simulink model "gfm_battery_sil"  (R2018b)
settings: Solver=ode45  StartTime=0.0  StopTime=100  RelTol=1e-3
PreLoadFcn:
  | load_system('../simulink_reference_models/test_sequence_lib');
  | load_system('../simulink_reference_models/controls_element_lib');
InitFcn:
  | close all;
  | clear all;
  | clc;
  | 
  | % frequency nominals
  | F_NOM = 60;
  | W_NOM = 2 * pi * F_NOM;
  | 
  | % base values relative to inverter
  | % --------------------------------
  | VLL_INV_NOM = 480;
  | P_INV_NOM = 1e6;
  | Q_INV_NOM = 0.5e6;
  | S_INV_NOM = sqrt(P_INV_NOM^2 + Q_INV_NOM^2);
  | 
  | I_INV_BASE = S_INV_NOM/(sqrt(3)*VLL_INV_NOM);
  | Z_INV_BASE = VLL_INV_NOM^2/S_INV_NOM;
  | L_INV_BASE = Z_INV_BASE / W_NOM;
  | C_INV_BASE = 1 / (Z_INV_BASE * W_NOM);
  | 
  | % nominal ratings for power system model
  | % --------------------------------------
  | INVERTER_COUNT = 100;
  | 
  | VLV_NOM = VLL_INV_NOM;
  | VMV_NOM = 35e3;
  | VHV_NOM = 230e3;
  | S_PLANT = INVERTER_COUNT * S_INV_NOM;
  | 
  | N_GSU = VHV_NOM/VMV_NOM;
  | N_MVT = VMV_NOM/VLV_NOM;
  | 
  | I_LV_BASE = S_PLANT/(sqrt(3)*VLV_NOM);
  | I_MV_BASE = S_PLANT/(sqrt(3)*VMV_NOM);
  | I_HV_BASE = S_PLANT/(sqrt(3)*VHV_NOM);
  | 
  | Z_LV_BASE = VLV_NOM^2/S_PLANT;
  | Z_MV_BASE = VMV_NOM^2/S_PLANT;
  | Z_HV_BASE = VHV_NOM^2/S_PLANT;
  | 
  | L_LV_BASE = Z_LV_BASE / W_NOM;
  | L_MV_BASE = Z_MV_BASE / W_NOM;
  | L_HV_BASE = Z_HV_BASE / W_NOM;
  | C_LV_BASE = 1 / (Z_LV_BASE * W_NOM);
  | C_MV_BASE = 1 / (Z_MV_BASE * W_NOM);
  | C_HV_BASE = 1 / (Z_HV_BASE * W_NOM);
libraries: test_sequence_lib x11, controls_element_lib x2
settings Model: SimulationMode=accelerator  Creator=HussamAlatrash  LastModifiedBy=ahhei
settings DataIOCC: ReturnWorkspaceOutputs=on
settings DebuggingCC: UnconnectedInputMsg=none  UnconnectedOutputMsg=none  UnconnectedLineMsg=none
settings ModelReferenceCC: EnableRefExpFcnMdlSchedulingChecks=off
settings RTWCC: Description=Generic Real-Time Target
settings ConfigComp: CovBoundaryAbsTol=1.0e-5

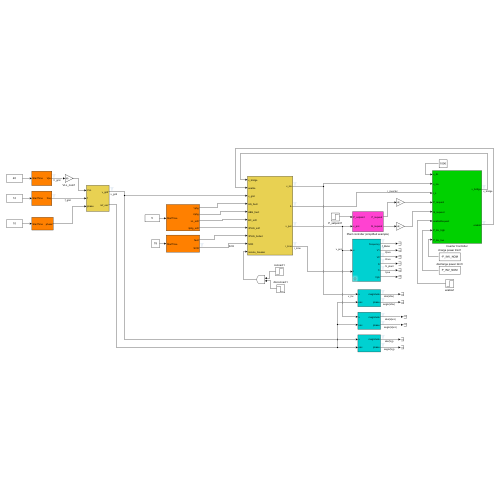
[thumbnail: Simulink's stored preview of the top-level diagram]
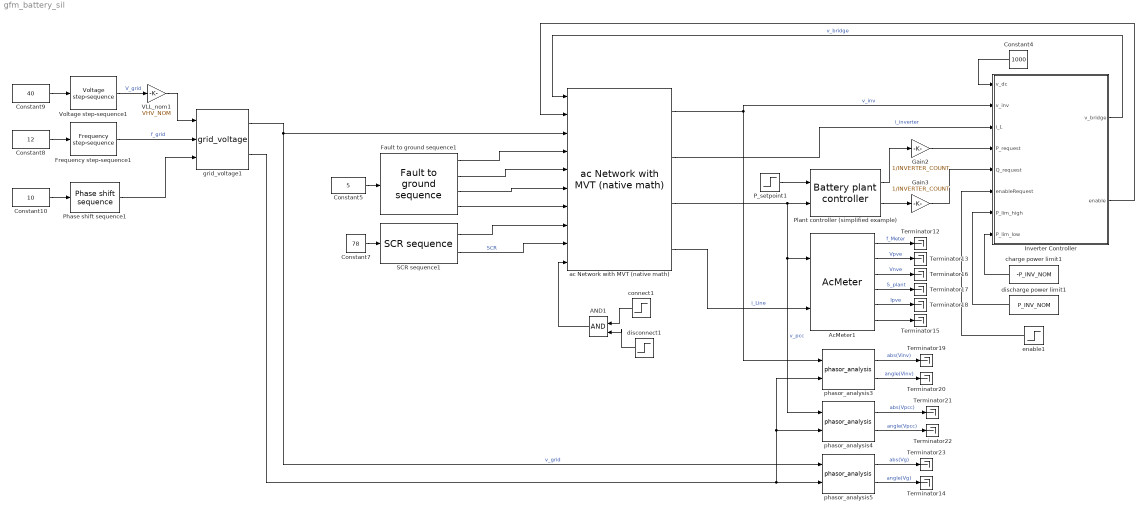
== system gfm_battery_sil ==
  AND1 : Logic  IconShape=distinctive  AllPortsSameDT=off  OutDataTypeStr=boolean
  AcMeter1 : test_sequence_lib/AcMeter  VllRated=VHV_NOM
  Constant10 : Constant  Value=10
  Constant4 : Constant  Value=1000
  Constant5 : Constant  Value=5
  Constant7 : Constant  Value=78
  Constant8 : Constant  Value=12
  Constant9 : Constant  Value=40
  Fault to ground sequence1 : test_sequence_lib/Fault to ground sequence  SystemSampleTime=-1  EmptyChoice=off  PassThrough=off  PassThroughVariantControl=(default)  EmptyChoiceVariantControl=(default)  Latency=0  AutoFrameSizeCalculation=off
  Frequency step-sequence1 : test_sequence_lib/Frequency step-sequence  SystemSampleTime=-1  EmptyChoice=off  PassThrough=off  PassThroughVariantControl=(default)  EmptyChoiceVariantControl=(default)  Latency=0  AutoFrameSizeCalculation=off
  Gain2 : Gain  Gain=1/INVERTER_COUNT
  Gain3 : Gain  Gain=1/INVERTER_COUNT
  Inverter Controller : Subsystem
  P_setpoint1 : Step  Time=4  After=S_PLANT*0.5  SampleTime=0
  Phase shift sequence1 : test_sequence_lib/Phase shift sequence  SystemSampleTime=-1  EmptyChoice=off  PassThrough=off  PassThroughVariantControl=(default)  EmptyChoiceVariantControl=(default)  Latency=0  AutoFrameSizeCalculation=off
  Plant controller (simplified example) : controls_element_lib/Battery plant controller  SystemSampleTime=-1  EmptyChoice=off  PassThrough=off  PassThroughVariantControl=(default)  EmptyChoiceVariantControl=(default)  Latency=0  AutoFrameSizeCalculation=off
  SCR sequence1 : test_sequence_lib/SCR sequence  SystemSampleTime=-1  EmptyChoice=off  PassThrough=off  PassThroughVariantControl=(default)  EmptyChoiceVariantControl=(default)  Latency=0  AutoFrameSizeCalculation=off
  Terminator{12..23} (12 alike) : Terminator
  VLL_nom1 : Gain  Gain=VHV_NOM
  Voltage step-sequence1 : test_sequence_lib/Voltage step-sequence  SystemSampleTime=-1  EmptyChoice=off  PassThrough=off  PassThroughVariantControl=(default)  EmptyChoiceVariantControl=(default)  Latency=0  AutoFrameSizeCalculation=off
  ac Network with MVT (native math) : test_sequence_lib/ac Network with MVT (native math)  SystemSampleTime=-1  EmptyChoice=off  PassThrough=off  PassThroughVariantControl=(default)  EmptyChoiceVariantControl=(default)  Latency=0  AutoFrameSizeCalculation=off
  charge power limit1 : Constant  Value=-P_INV_NOM
  connect1 : Step  Time=0  SampleTime=0
  discharge power limit1 : Constant  Value=P_INV_NOM
  disconnect1 : Step  Time=97  Before=1  After=0  SampleTime=0
  enable1 : Step  Time=0.5  SampleTime=0
  grid_voltage1 : test_sequence_lib/grid_voltage  SystemSampleTime=-1  EmptyChoice=off  PassThrough=off  PassThroughVariantControl=(default)  EmptyChoiceVariantControl=(default)  Latency=0  AutoFrameSizeCalculation=off
  phasor_analysis3 : test_sequence_lib/phasor_analysis  SystemSampleTime=-1  EmptyChoice=off  PassThrough=off  PassThroughVariantControl=(default)  EmptyChoiceVariantControl=(default)  Latency=0  AutoFrameSizeCalculation=off
  phasor_analysis4 : test_sequence_lib/phasor_analysis  SystemSampleTime=-1  EmptyChoice=off  PassThrough=off  PassThroughVariantControl=(default)  EmptyChoiceVariantControl=(default)  Latency=0  AutoFrameSizeCalculation=off
  phasor_analysis5 : test_sequence_lib/phasor_analysis  SystemSampleTime=-1  EmptyChoice=off  PassThrough=off  PassThroughVariantControl=(default)  EmptyChoiceVariantControl=(default)  Latency=0  AutoFrameSizeCalculation=off
  wires:
  Voltage step-sequence1/1 -> VLL_nom1/1  "V_grid"
  Constant9/1 -> Voltage step-sequence1/1
  Fault to ground sequence1/2 -> ac Network with MVT (native math)/5
  AND1/1 -> ac Network with MVT (native math)/10
  Constant4/1 -> Inverter Controller/1(v_dc)
  Constant10/1 -> Phase shift sequence1/1
  AcMeter1/3 -> Terminator16/1  "Vnve"
  discharge power limit1/1 -> Inverter Controller/7(P_lim_high)
  Fault to ground sequence1/3 -> ac Network with MVT (native math)/6
  AcMeter1/6 -> Terminator15/1
  Inverter Controller/1(v_bridge) -> ac Network with MVT (native math)/1  "v_bridge"
  Constant7/1 -> SCR sequence1/1
  AcMeter1/2 -> Terminator13/1  "Vpve"
  Plant controller (simplified example)/1 -> Gain2/1
  ac Network with MVT (native math)/1 -> Inverter Controller/2(v_inv), phasor_analysis3/1  "v_inv"
  Constant5/1 -> Fault to ground sequence1/1
  P_setpoint1/1 -> Plant controller (simplified example)/1
  phasor_analysis5/1 -> Terminator23/1  "abs(Vg)"
  AcMeter1/5 -> Terminator18/1  "Ipve"
  Gain3/1 -> Inverter Controller/5(Q_request)
  Plant controller (simplified example)/2 -> Gain3/1
  grid_voltage1/1 -> ac Network with MVT (native math)/3, phasor_analysis5/1  "v_grid"
  phasor_analysis4/2 -> Terminator22/1  "angle(Vpcc)"
  SCR sequence1/1 -> ac Network with MVT (native math)/8
  phasor_analysis3/1 -> Terminator19/1  "abs(Vinv)"
  Phase shift sequence1/1 -> grid_voltage1/3
  AcMeter1/4 -> Terminator17/1  "S_plant"
  ac Network with MVT (native math)/4 -> AcMeter1/2  "i_Line"
  AcMeter1/1 -> Terminator12/1  "f_Meter"
  VLL_nom1/1 -> grid_voltage1/1
  phasor_analysis3/2 -> Terminator20/1  "angle(Vinv)"
  SCR sequence1/2 -> ac Network with MVT (native math)/9  "SCR"
  ac Network with MVT (native math)/2 -> Inverter Controller/3(i_L)  "i_inverter"
  disconnect1/1 -> AND1/2
  Fault to ground sequence1/4 -> ac Network with MVT (native math)/7
  Gain2/1 -> Inverter Controller/4(P_request)
  ac Network with MVT (native math)/3 -> Plant controller (simplified example)/2, phasor_analysis4/1, AcMeter1/1  "v_pcc"
  charge power limit1/1 -> Inverter Controller/8(P_lim_low)
  Inverter Controller/2(enable) -> ac Network with MVT (native math)/2
  Frequency step-sequence1/1 -> grid_voltage1/2  "f_grid"
  Fault to ground sequence1/1 -> ac Network with MVT (native math)/4
  phasor_analysis4/1 -> Terminator21/1  "abs(Vpcc)"
  grid_voltage1/2 -> phasor_analysis4/2, phasor_analysis3/2, phasor_analysis5/2
  phasor_analysis5/2 -> Terminator14/1  "angle(Vg)"
  enable1/1 -> Inverter Controller/6(enableRequest)
  connect1/1 -> AND1/1
  Constant8/1 -> Frequency step-sequence1/1

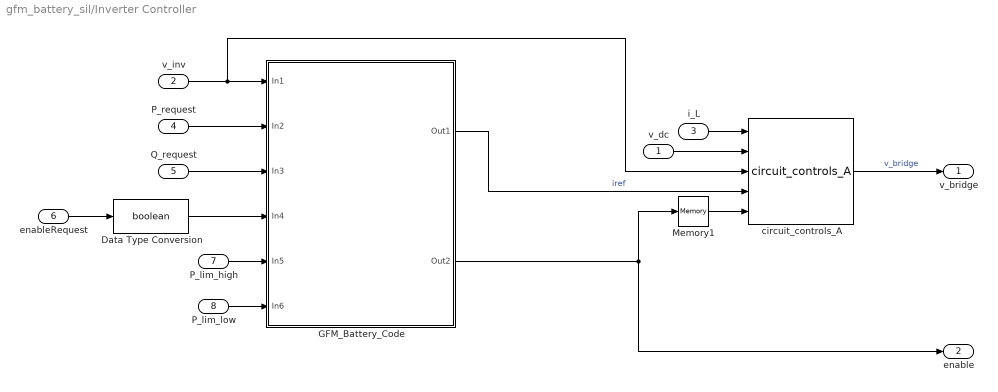
== system gfm_battery_sil/Inverter Controller ==
  v_dc : Inport
  v_inv : Inport  Port=2
  i_L : Inport  Port=3
  P_request : Inport  Port=4
  Q_request : Inport  Port=5
  enableRequest : Inport  Port=6
  P_lim_high : Inport  Port=7
  P_lim_low : Inport  Port=8
  Data Type Conversion : DataTypeConversion  OutDataTypeStr=boolean
  GFM_Battery_Code : Subsystem  Description=Replaced Block  mask(Replaced Block){}
      mask help: This block has been replaced with an empty subsystem because it used functionality that is unavailable in Simulink R2018b.
      mask Display: fprintf('Replaced: %s\n','CFunction')
  Memory1 : Memory
  circuit_controls_A : controls_element_lib/circuit_controls_A  SystemSampleTime=-1  EmptyChoice=off  PassThrough=off  PassThroughVariantControl=(default)  EmptyChoiceVariantControl=(default)  Latency=0  AutoFrameSizeCalculation=off
  v_bridge : Outport
  enable : Outport  Port=2
  wires:
  GFM_Battery_Code/1(Out1) -> circuit_controls_A/4  "iref"
  v_dc/1 -> circuit_controls_A/2
  circuit_controls_A/1 -> v_bridge/1  "v_bridge"
  i_L/1 -> circuit_controls_A/1
  Q_request/1 -> GFM_Battery_Code/3(In3)
  P_request/1 -> GFM_Battery_Code/2(In2)
  P_lim_low/1 -> GFM_Battery_Code/6(In6)
  P_lim_high/1 -> GFM_Battery_Code/5(In5)
  v_inv/1 -> GFM_Battery_Code/1(In1), circuit_controls_A/3
  Memory1/1 -> circuit_controls_A/5
  enableRequest/1 -> Data Type Conversion/1
  GFM_Battery_Code/2(Out2) -> enable/1, Memory1/1
  Data Type Conversion/1 -> GFM_Battery_Code/4(In4)

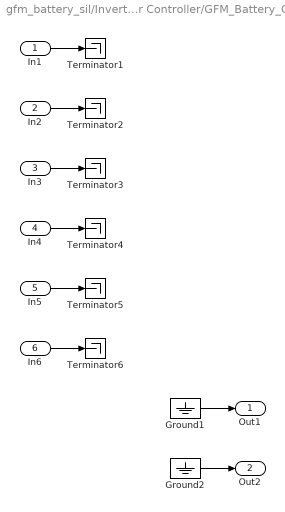
== system gfm_battery_sil/Inverter Controller/GFM_Battery_Code ==
  In1 : Inport
  In2 : Inport  Port=2
  In3 : Inport  Port=3
  In4 : Inport  Port=4
  In5 : Inport  Port=5
  In6 : Inport  Port=6
  Ground1 : Ground
  Ground2 : Ground
  Terminator{1..6} (6 alike) : Terminator
  Out1 : Outport
  Out2 : Outport  Port=2
  wires:
  Ground2/1 -> Out2/1
  Ground1/1 -> Out1/1
  In6/1 -> Terminator6/1
  In5/1 -> Terminator5/1
  In4/1 -> Terminator4/1
  In3/1 -> Terminator3/1
  In2/1 -> Terminator2/1
  In1/1 -> Terminator1/1
